simulink model "hrg_v10_electrical_only"  (R2025a)
settings: Solver=FixedStepDiscrete  StartTime=0.0  StopTime=p.duration  FixedStep=p.Ts  RelTol=1e-3
model workspace (MAT data in the model file):
  Ad = [0.987688404648  0  2.48971240774e-05  0  2.3550629281e-16  0  -1.05053344817e-16  0  -1.37851257349e-17  0  0  0; 0  0.987688404601  0  2.48971241759e-05  0  2.35506727885e-16  0  -1.10320415602e-16  0  -1.37851257347e-17  0  0; -982.899001252  0  0.987672737453  0  1.56117115743e-11  0  1.04722997195e-12  0  6.69881883777e-15  0  0  0; 0  -982.899001238  0  0.987672737407  0  1.56117113326e-11  0  1.05221738801e-12  0  6.69881883773e-15  0  0; 0  0  0  0  0.28650479686  0  0  0  0  0  0  0; 0  0  0  0  0  0.28650479686  0  0  0  0  0  0; 943869.86657  0  -988.617130528  0  -2.27745303207e-06  0  -1.02941392962e-09  0  -6.18034740695e-12  0  0  0; 0  943869.866557  0  -988.617130486  0  -2.27745303184e-06  0  -1.03419322393e-09  0  -6.18034740691e-12  0  0; 113668107.874  0  -239056.237719  0  -0.00104980715024  0  9.99759911472  0  0.999750030756  0  0  0; 0  113668107.873  0  -239056.237716  0  -0.00104980715023  0  9.99759911417  0  0.999750030756  0  0; 62170959.0903  0  -163920.515662  0  -0.000798963915782  0  9.50410730835  0  0.956612237543  0  0.0432139182638  0; 0  62170959.0901  0  -163920.515661  0  -0.000798963915774  0  9.50410730805  0  0.956612237543  0  0.0432139182638]
  Bd = [1.07535202977e-16  0; 0  1.07534912816e-16; 1.17750951158e-11  0; 0  1.17750952858e-11; 0.71349520314  0; 0  0.71349520314; 2.25115370575e-06  0; 0  2.25115370559e-06; 0.00104663998201  0; 0  0.001046639982; 0.000797231627893  0; 0  0.000797231627887]
  p.f0 = 1000.00000005
  p.gamma = 0.31415877964
  p.Cs = 1.00000000606e-09
  p.G0 = 1.00131870607e-10
  p.kappa = 9.99998939716e-07
  p.b = 1.09999886801e-06
  p.Cds = 1.50018875063e-13
  p.Ts = 2.5e-05
  p.Tc = 0.001
  p.duration = 0.6
  p.Omega = 0
  p.B = []
  p.charge_target_C = 1e-11
  p.alpha0 = 0.4
  p.driver_tau = 2e-05
  p.Cf = 1e-10
  p.Rf = 1000000000
  p.afe_bw = 20000
  p.adc_span = 2
  p.adc_bits = 20
  p.dac_span = 2
  p.dac_bits = 18
  p.vmax = 1
  p.agc_bw = 5
  p.quad_bw = 4
  p.pll_gain = 30
  p.max_detune = 30
  p.gain_y = 1
  p.calibrate = 1
  p.synthetic = 1
  p.Rs = 1000
  x0 = [2.76318298201e-12; 1.16825502693e-12; 0; 0; 0; 0; 0; 0; 0; 0; 0; 0]
Description:
  | Electrical-only synthetic research model. States 1:2 are motional charge [C], NOT displacement [m]. No mass, Theta or B supplied for stationary test.
settings Model: Creator=11725  LastModifiedBy=11725

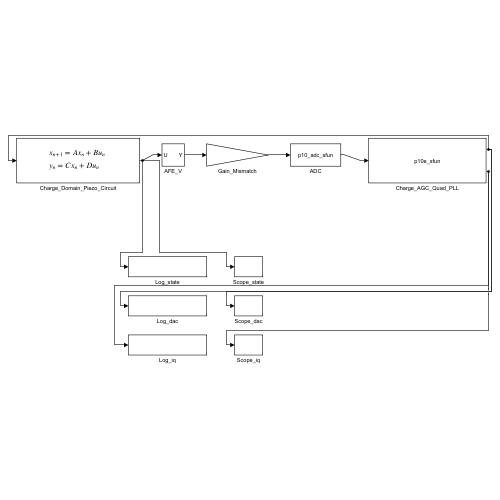
[thumbnail: Simulink's stored preview of the top-level diagram]
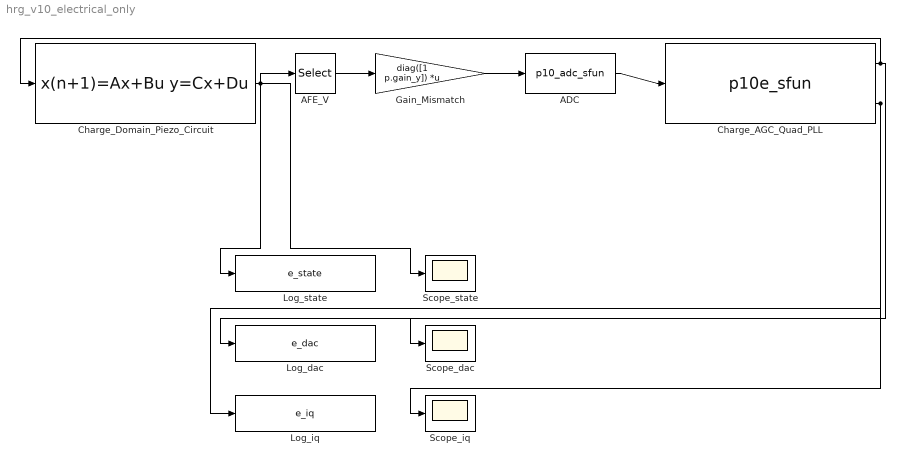
== system hrg_v10_electrical_only ==
  ADC : M-S-Function  FunctionName=p10_adc_sfun  Parameters=p
  AFE_V : Selector  InputPortWidth=12  IndexOptions=Index vector (dialog)  Indices=[11 12]  OutputSizes=1
  Charge_AGC_Quad_PLL : M-S-Function  FunctionName=p10e_sfun  Parameters=p
  Charge_Domain_Piezo_Circuit : DiscreteStateSpace  A=Ad  B=Bd  C=eye(12)  D=zeros(12,2)  InitialCondition=x0  SampleTime=p.Ts
  Gain_Mismatch : Gain  Gain=diag([1 p.gain_y])  Multiplication=Matrix(K*u)
  Log_dac : ToWorkspace  VariableName=e_dac  SaveFormat=Timeseries  SampleTime=-1
  Log_iq : ToWorkspace  VariableName=e_iq  SaveFormat=Timeseries  SampleTime=-1
  Log_state : ToWorkspace  VariableName=e_state  SaveFormat=Timeseries  SampleTime=-1
  Scope_dac : Scope
  Scope_iq : Scope
  Scope_state : Scope
  wires:
  Charge_Domain_Piezo_Circuit/1 -> AFE_V/1, Log_state/1, Scope_state/1
  AFE_V/1 -> Gain_Mismatch/1
  Gain_Mismatch/1 -> ADC/1
  ADC/1 -> Charge_AGC_Quad_PLL/1
  Charge_AGC_Quad_PLL/1 -> Charge_Domain_Piezo_Circuit/1, Log_dac/1, Scope_dac/1
  Charge_AGC_Quad_PLL/2 -> Log_iq/1, Scope_iq/1
